simulink model "Controlador_LQR_PIL"  (R2026b)
settings: Solver=FixedStepDiscrete  StopTime=inf  FixedStep=Ts  EnableMultiTasking=on
InitFcn:
  | init_BOOT
values from neighbouring files (symbols this model uses):
  Ki_LQR = K_LQR(3)    [init_BOOT.m]
  Ku_LQR = K_LQR(2)    [init_BOOT.m]
  Kx_LQR = K_LQR(1)    [init_BOOT.m]
  Ts = evalin('base', 'Ts')    [ejecutar_PIL.m]    (also in init_BOOT.m = 0.00025; prueba_independencia_PIL.m)
undefined symbols (not defined in the file or in its folder): DiscIntNeverNeededParam
settings Model: SILPILModeSetting=veronly  Creator=Usuario  LastModifiedBy=matia
settings SolverCC: AutoInsertRateTranBlk=on
settings DataIOCC: SaveOutput=off  SaveTime=off
settings OptimizationCC: DifferentSizesBufferReuse=on  EfficientTunableParamExpr=on  EnhancedBackFolding=on  MaxStackSize=64  OptimizationCustomize=off  OptimizeBlockOrder=speed  PassReuseOutputArgsAs=Individual arguments
settings DebuggingCC: ParameterTunabilityLossMsg=error
settings HardwareCC: ProdHWDeviceType=Atmel->AVR  ProdLargestAtomicFloat=None
settings ModelReferenceCC: PropagateVarSize=During execution
settings SFSimCC: MATLABDynamicMemAlloc=off
settings RTWCC: BuildConfiguration=Faster Runs  Description=Embedded Coder  HardwareBoard=Arduino Mega 2560  SystemTargetFile=ert.tlc  TLCOptions=-aInlineSetEventsForThisBaseRateFcn=TLC_FALSE -aSuppressMultiTaskScheduler=TLC_FALSE -aRateBasedStepFcn=1  TemplateMakefile=ert_default_tmf  Toolchain=Arduino AVR
settings CodeAppCC: ForceParamTrailComments=on  IgnoreCustomStorageClasses=off  InsertBlockDesc=on  OperatorAnnotations=on  SFDataObjDesc=on  SimulinkDataObjDesc=on
settings ERTTargetCC: CodeInterfacePackaging=Reusable function  ExtModeAutomaticAllocSize=off  ExtModeIntrfLevel=Level2 - Open  ExtModeMexFile=ext_xcp  ExtModeStaticAlloc=on  RootIOFormat=Structure reference  SupportContinuousTime=on  SupportVariableSizeSignals=on

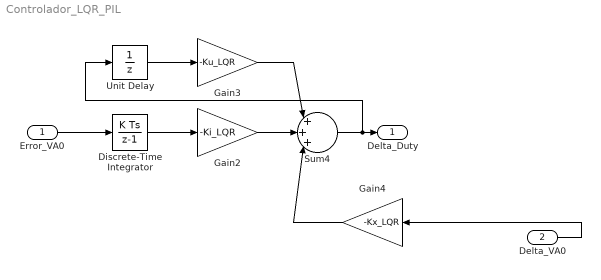
== system Controlador_LQR_PIL ==
  Error_VA0 : Inport  OutDataTypeStr=single  PortDimensions=1  SampleTime=[0.00025000000000000001,0]
  Delta_VA0 : Inport  Port=2  OutDataTypeStr=single  PortDimensions=1  SampleTime=[0.00025000000000000001,0]
  Discrete-Time Integrator : DiscreteIntegrator  SampleTime=Ts  OutDataTypeStr=single  ICPrevOutput=DiscIntNeverNeededParam  ICPrevScaledInput=DiscIntNeverNeededParam
  Gain2 : Gain  Gain=-Ki_LQR  OutDataTypeStr=Inherit: Same as input  ParamDataTypeStr=Inherit: Same as input
  Gain3 : Gain  Gain=-Ku_LQR  OutDataTypeStr=Inherit: Same as input  ParamDataTypeStr=Inherit: Same as input
  Gain4 : Gain  Gain=-Kx_LQR  OutDataTypeStr=Inherit: Same as input  ParamDataTypeStr=Inherit: Same as input
  Sum4 : Sum  Inputs=|+++|  OutDataTypeStr=single
  Unit Delay : UnitDelay  SampleTime=Ts
  Delta_Duty : Outport  OutDataTypeStr=single  PortDimensions=1  SampleTime=[0.00025000000000000001,0]
  wires:
  Unit Delay/1 -> Gain3/1
  Discrete-Time Integrator/1 -> Gain2/1
  Delta_VA0/1 -> Gain4/1
  Gain3/1 -> Sum4/1
  Gain2/1 -> Sum4/2
  Gain4/1 -> Sum4/3
  Sum4/1 -> Delta_Duty/1, Unit Delay/1
  Error_VA0/1 -> Discrete-Time Integrator/1
